simulink model "BasicRobotV3Animation"  (R2025b)
settings: Solver=VariableStepAuto  StartTime=0.0  StopTime=50.0  RelTol=1e-3
PreLoadFcn:
  | BasicRobot_Parameters
InitFcn:
  | BasicRobot_Parameters
undefined symbols (not defined in the file): m, magnitude, r, r_ref, theta0, theta_ref, v_ref, x_obs, y_obs
libraries: sim3dlib x3
settings Model: Creator=BeanieBabyJ  LastModifiedBy=AORUS
settings SolverCC: ZeroCrossAlgorithm=Adaptive
settings DebuggingCC: IgnoredZcDiagnostic=none
settings RTWCC: GPUComputeCapability=3.5

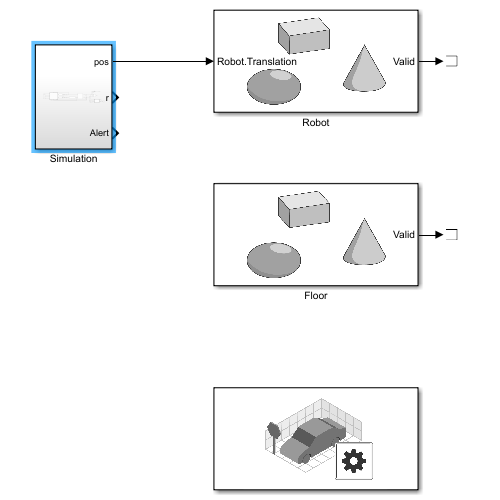
[thumbnail: Simulink's stored preview of the top-level diagram]
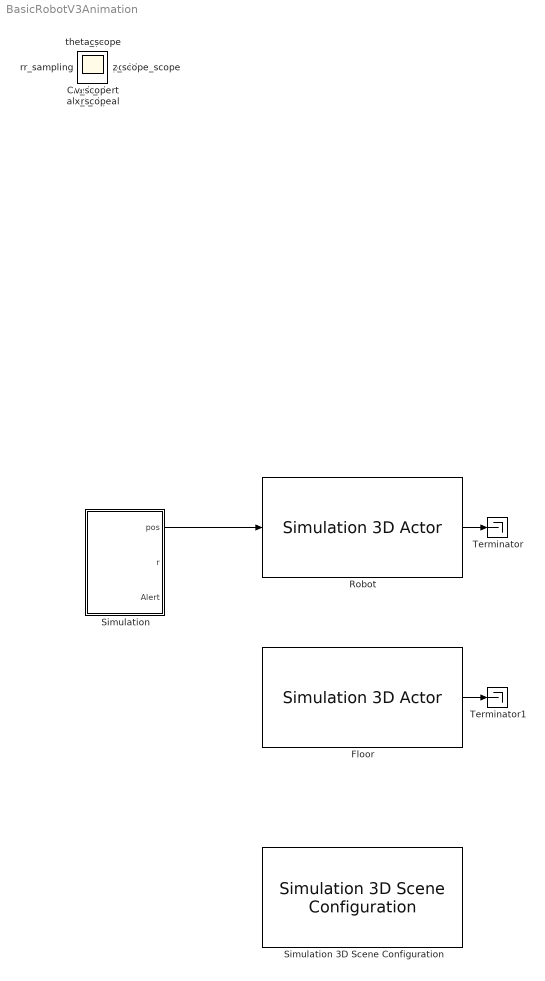
== system BasicRobotV3Animation ==
  Floor : sim3dlib/Simulation 3D Actor  Priority=1  ActorName=Floor  ParentName=Scene Origin  Operation=Create at setup  InitScriptText=|  SampleTime=-1  Translation=[0 0 0]  Rotation=[0 0 0]  Scale=[1 1 1]  aMode=5  ActorTag=Floor  ActorType=Sim3dActor  ID=C
      | createShape(Actor,'plane', [5 5 0.1]);
      | Actor.PreciseContacts = true;
  Robot : sim3dlib/Simulation 3D Actor  Priority=1  ActorName=Robot  ParentName=Scene Origin  Operation=Create at setup  InitScriptText=|  SampleTime=-1  Translation=[0 0 0.25]  Rotation=[0 0 0]  Scale=[1 1 1]  InputsText=Robot.Translation  aMode=5  ActorTag=Robot  ActorType=Sim3dActor  ID=C
      | createShape(Actor,'cylinder',[1 1 0.25]);
      | Actor.Color = [0 0 1];
  Simulation : Subsystem
  Simulation 3D Scene Configuration : sim3dlib/Simulation 3D Scene Configuration  Priority=0  ProjectFormat=Default Scenes  SceneDesc=Empty scene  ProjectName=C:\Program Files\MATLAB\R2025b\toolbox\shared\sim3d_projects\automotive_project_windows\UE\WindowsNoEditor\VehicleSimulation.exe  ScenePath=/Game/Maps/HwStrght  EnableOpenDRIVE=off  vehTagList={'Custom';'Robot';'Scene Origin'}  vehTag=Scene Origin  AttachedCameraRelativeTranslation=[0 0 0]  FreeCameraDefaultInitialTranslation=[-6, 0, 2]  AttachedCameraRelativeRotation=[0 0 0]  FreeCameraDefaultInitialRotation=[0, -15, 0]  ViewpointName=Custom  FreeCameraInitialTranslation=[0 0 0]  ViewpointTranslation=[0 0 0]  FreeCameraInitialRotation=[0 0 0]  ViewpointRotation=[0 0 0]  OpVisEn=off  Ts=.02  EnableWindow=on  EnableRemoteAccess=off  EnableWeather=off  SunAzimuth=90  SunAltitude=40.0  EnableGeospatialSun=off  Latitude=0  Longitude=0  Date=2023-01-01  Time=10:30:00  GeoTimeZone=-5.0  SunDaylightSaving=off  wind=1  clouds=10  EnableVolumetricClouds=off  CloudCoverage=0  CloudAltitude=6  fog=0  rain=0  RaindropsEffect=off  SnowDensity=0  EnableGeospatial=off  TilesetSource=Earth terrain  UseTrueOrigin=off  OriginHeight=200  OriginLatitude=40.744652  OriginLongitude=-73.988864  MapStyle=Aerial  AdditionalAssetIDs=[]  UseAdvancedSunSky=off  SolarTime=11  TimeZone=-5  Day=21  Month=9  Year=2022  UseDaylightSavingTime=on  DSTStartDay=10  DSTStartMonth=3  DSTEndDay=3  DSTEndMonth=11  DSTSwitchHour=2  sensorTag=MainCamera1  sensorId=1  sensorName=MainCamera1  mountLoc=Origin  offsetFlag=off  tmountOffset=[0, 0, 0]  rmountOffset=[0, 0, 0]  HorizontalResolution=1280  VerticalResolution=720  HorizontalFOV=60  mountPoint=[0 0 0]  mountOrientation=[0 0 0]  aMode=5  ID=1  GeoTrigger=Inactive  ViewNameList={'Custom'}  ViewTranslationList={'[0 0 0]'}  ViewRotationList={'[0 0 0]'}
      settings: LibrarySourceBlock=sl3dlib/Simulation 3D/Environment/Simulation 3D Scene Configuration
  Terminator : Terminator
  Terminator1 : Terminator
  Crash_alert : Scope
      settings: ActiveDisplayYMinimum=-1  ActiveDisplayYMaximum=1  DataLoggingVariableName=ScopeData5
  Scope : Scope
      settings: ActiveDisplayYMinimum=-0.81338  ActiveDisplayYMaximum=3.46533
  alert_signal : Scope
      settings: ActiveDisplayYMinimum=-1  ActiveDisplayYMaximum=1  DataLoggingVariableName=ScopeData5
  position_scope : Scope
      settings: ActiveDisplayYMinimum=-0.58155  ActiveDisplayYMaximum=5.23399
  rr_sampling : Scope
      settings: ActiveDisplayYMinimum=-0.42527  ActiveDisplayYMaximum=3.82747
  theta_scope : Scope
      settings: ActiveDisplayYMinimum=-0.21049  ActiveDisplayYMaximum=1.89437  DataLoggingVariableName=ScopeData3
  v_scope : Scope
      settings: ActiveDisplayYMinimum=-0.0225  ActiveDisplayYMaximum=0.2025  DataLoggingVariableName=ScopeData2
  x_scope : Scope
      settings: ActiveDisplayYMinimum=-0.35975  ActiveDisplayYMaximum=3.23772
  z_scope : Scope
      settings: ActiveDisplayYMinimum=-0.22681  ActiveDisplayYMaximum=2.04125
  wires:
  Simulation/1(pos) -> Robot/1
  Robot/1 -> Terminator/1
  Floor/1 -> Terminator1/1

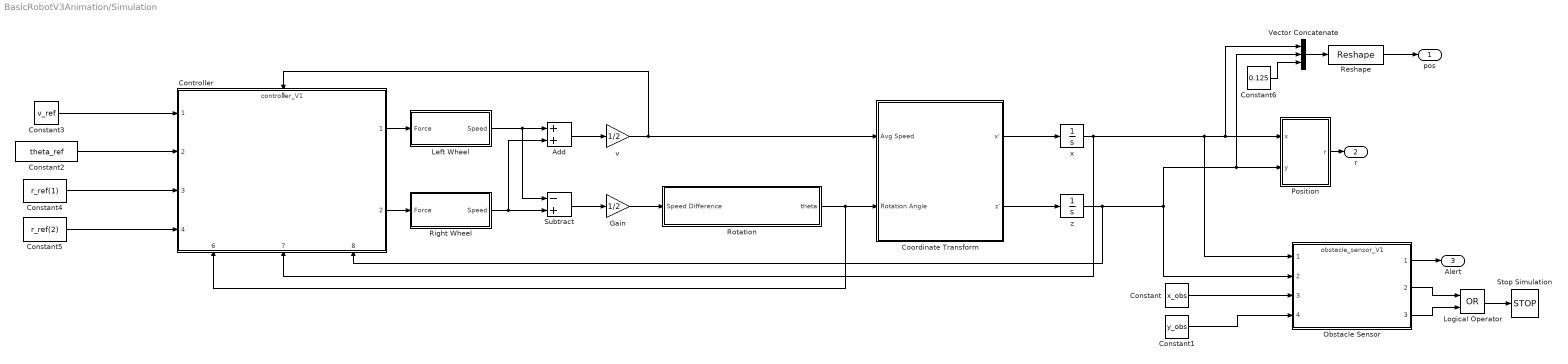
== system BasicRobotV3Animation/Simulation ==
  Add : Sum
  Constant : Constant  Value=x_obs
  Constant1 : Constant  Value=y_obs
  Constant2 : Constant  Value=theta_ref
  Constant3 : Constant  Value=v_ref
  Constant4 : Constant  Value=r_ref(1)
  Constant5 : Constant  Value=r_ref(2)
  Constant6 : Constant  Value=0.125
  Controller : ModelReference  ModelNameDialog=controller_V1  SimulationMode=Normal  ModelReferenceVersion=1.1
      settings: PortSchema="{\"entries\":[{\"content\":{\"sides\":[{\"content\":{\"connectorIds\":[\"In1\",\"In2\",\"In3\",\"In4\"]},\"type\":\"ConnectorPlacement.EquallySpacedRectSide\",\"uuid\":\"77adb04a-7511-4a05-94fb-1165319a2d74\"},{\"content\":{\"connectorIds\":[\"Out1\",\"Out2\"],\"side\":\"RIGHT\"},\"type\":\"ConnectorPlacement.EquallySpacedRectSide\",\"uuid\":\"b527b03e-d73b-4ce6-867f-ec77326eb6a4\"},{\"content\":{\"connectorIds\":[\"In5\"],\"side\":\"TOP\"},\"type\":\"ConnectorPlacement.EquallySpacedRectSide\",\"uuid\":\"f209cd25-4a1c-4c4c-8152-827ba43394a2\"},{\"content\":{\"connectorIds\":[\"In6\",\"In7\",\"In8\"],\"side\":\"BOTTOM\"},\"type\":\"ConnectorPlacement.EquallySpacedRectSide\",\"uuid\":\"fa4cf634-6de0-464d-8748-7f9791395bbd\"}]},\"type\":\"ConnectorPlacement.EquallySpacedConnector\",\"uuid\":\"5619af3e-39e8-40d6-a89c-5a796356accd\"}],\"packageUris\":[\"http://schema.mathworks.com/mf0/Connector/R2020b\"],\"version\":\"1.0\"}"
  Coordinate Transform : Subsystem
  Gain : Gain  Gain=1/2
  Left Wheel : Subsystem
  Logical Operator : Logic  Operator=OR  AllPortsSameDT=off  OutDataTypeStr=boolean
  Obstacle Sensor : ModelReference  ModelNameDialog=obstacle_sensor_V1  SimulationMode=Normal  ModelReferenceVersion=1.1
  Position : Subsystem
  Reshape : Reshape  OutputDimensionality=Row vector (2-D)
  Right Wheel : Subsystem
  Rotation : Subsystem
  Stop Simulation : Stop
  Subtract : Sum  Inputs=-+
  Vector Concatenate : Concatenate  NumInputs=3
  v : Gain  Gain=1/2
  x : Integrator
  z : Integrator
  pos : Outport
  r : Outport  Port=2
  Alert : Outport  Port=3
  wires:
  Gain/1 -> Rotation/1(Speed Difference)
  Right Wheel/1(Speed) -> Add/2, Subtract/2
  z/1 -> Controller/8, Obstacle Sensor/2, Vector Concatenate/2, Position/2(y)
  Position/1(r) -> r/1
  Add/1 -> v/1
  Rotation/1(theta) -> Controller/6, Coordinate Transform/2(Rotation Angle)
  Constant5/1 -> Controller/4
  Subtract/1 -> Gain/1
  Constant4/1 -> Controller/3
  x/1 -> Controller/7, Obstacle Sensor/1, Vector Concatenate/1, Position/1(x)
  Logical Operator/1 -> Stop Simulation/1
  Coordinate Transform/1(x') -> x/1
  Vector Concatenate/1 -> Reshape/1
  Obstacle Sensor/3 -> Logical Operator/2
  Controller/2 -> Right Wheel/1(Force)
  Left Wheel/1(Speed) -> Add/1, Subtract/1
  Constant2/1 -> Controller/2
  Constant/1 -> Obstacle Sensor/3
  Obstacle Sensor/1 -> Alert/1
  v/1 -> Controller/5, Coordinate Transform/1(Avg Speed)
  Coordinate Transform/2(z') -> z/1
  Controller/1 -> Left Wheel/1(Force)
  Constant3/1 -> Controller/1
  Constant1/1 -> Obstacle Sensor/4
  Obstacle Sensor/2 -> Logical Operator/1
  Constant6/1 -> Vector Concatenate/3
  Reshape/1 -> pos/1

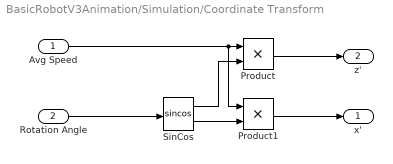
== system BasicRobotV3Animation/Simulation/Coordinate Transform ==
  Avg Speed : Inport
  Rotation Angle : Inport  Port=2
  Product : Product
  Product1 : Product
  SinCos : Trigonometry  Operator=sincos
  x' : Outport
  z' : Outport  Port=2
  wires:
  Rotation Angle/1 -> SinCos/1
  Avg Speed/1 -> Product1/1, Product/1
  SinCos/1 -> Product/2
  SinCos/2 -> Product1/2
  Product/1 -> z'/1
  Product1/1 -> x'/1

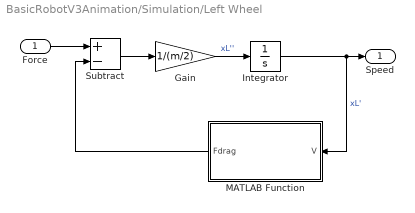
== system BasicRobotV3Animation/Simulation/Left Wheel ==
  Force : Inport
  Gain : Gain  Gain=1/(m/2)
  Integrator : Integrator
  MATLAB Function : MATLAB Function  TreatAsAtomicUnit=on
  Subtract : Sum  Inputs=+-
  Speed : Outport
  wires:
  Force/1 -> Subtract/1
  MATLAB Function/1(Fdrag) -> Subtract/2
  Subtract/1 -> Gain/1
  Integrator/1 -> MATLAB Function/1(V), Speed/1  "xL'"
  Gain/1 -> Integrator/1  "xL''"

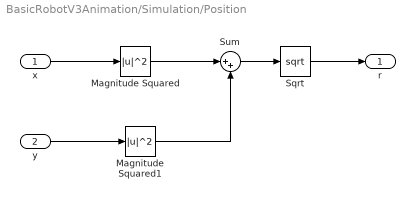
== system BasicRobotV3Animation/Simulation/Position ==
  x : Inport
  y : Inport  Port=2
  Magnitude Squared : Math  Operator=magnitude^2
  Magnitude Squared1 : Math  Operator=magnitude^2
  Sqrt : Sqrt
  Sum : Sum  Inputs=|++
  r : Outport
  wires:
  Magnitude Squared1/1 -> Sum/2
  Sum/1 -> Sqrt/1
  Magnitude Squared/1 -> Sum/1
  Sqrt/1 -> r/1
  x/1 -> Magnitude Squared/1
  y/1 -> Magnitude Squared1/1

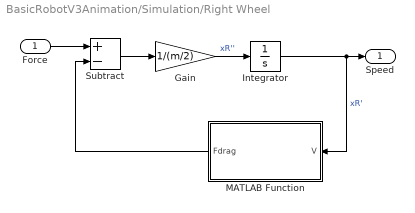
== system BasicRobotV3Animation/Simulation/Right Wheel ==
  Force : Inport
  Gain : Gain  Gain=1/(m/2)
  Integrator : Integrator
  MATLAB Function : MATLAB Function  TreatAsAtomicUnit=on
  Subtract : Sum  Inputs=+-
  Speed : Outport
  wires:
  Integrator/1 -> MATLAB Function/1(V), Speed/1  "xR'"
  Gain/1 -> Integrator/1  "xR''"
  Force/1 -> Subtract/1
  MATLAB Function/1(Fdrag) -> Subtract/2
  Subtract/1 -> Gain/1

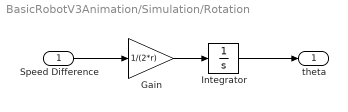
== system BasicRobotV3Animation/Simulation/Rotation ==
  Speed Difference : Inport
  Gain : Gain  Gain=1/(2*r)
  Integrator : Integrator  InitialCondition=theta0
  theta : Outport
  wires:
  Speed Difference/1 -> Gain/1
  Gain/1 -> Integrator/1
  Integrator/1 -> theta/1

== matlab function BasicRobotV3Animation/Simulation/Right Wheel/MATLAB Function ==
  data: Fdrag output; V input; k_drag parameter
function Fdrag=get_fdrag(V, k_drag)

Fdrag=k_drag*V*abs(V);

== matlab function BasicRobotV3Animation/Simulation/Left Wheel/MATLAB Function ==
  data: Fdrag output; V input; k_drag parameter
function Fdrag=get_fdrag(V, k_drag)

Fdrag=k_drag*V*abs(V);
